simulink model "RobustFormationControl_IntegerModel_under_Dis"  (R2023a)
settings: Solver=ode3  StartTime=0.0  StopTime=30  FixedStep=0.0001  RelTol=1e-3
InitFcn:
  | % % Parameters for the fractional order NTFSMC:
  | % Sliding Surface " Sx, Sy, and Sz ":
  | %------------------------
  | % 10
  | % 10
  | cx = 2*[4 4 4];
  | cxx = 1*[0.01 0.01 0.01];
  | 
  | cx1 = cx(1);
  | cy1 = cx(2);
  | cz1 = cx(3);
  | 
  | cx2 = cxx(1);
  | cy2 = cxx(2);
  | cz2 = cxx(3);
  | 
  | alpha1 = [0.6 0.6 0.6];
  | alpha2 = [0.1 0.1 0.1];
  | 
  | gammaX = [3 3 3];
  | gx  = gammaX(1);
  | gy = gammaX(2);
  | gz = gammaX(3);
  | 
  | p = 10;
  | q = 10;
  | 
  | % Sliding Surface " S_Phi , S_Theta, and  S_Psi":
  | %------------------------
  | cP = 2*[4 4 4];
  | cPP = 1*[0.01 0.01 0.01 0.01];
  | 
  | cPhi1 = cP(1);
  | cTheta1 = cP(2);
  | cPsi1 = cP(3);
  | 
  | cPhi2 = cPP(1);
  | cTheta2 = cPP(2);
  | cPsi2 = cPP(3);
  | gammaP = [3 3 3];
  | 
  | %=========================
  | %=========================
  | SigmaX = 1*[0.01 0.01 0.01];
  | SigmaXX =1*[1 1 1];
  | 
  | Sigma1X = SigmaX(1);
  | Sigma1Y = SigmaX(2);
  | Sigma1Z = SigmaX(3);
  | %-----
  | Sigma2X = SigmaXX(1);
  | Sigma2Y = SigmaXX(2);
  | Sigma2Z = SigmaXX(3);
  | 
  | 
  | SigmaP = 1*[0.01 0.01 0.01];
  | SigmaPP =1*[1 1 1];
  | 
  | Sigma1Phi   = SigmaP(1);
  | Sigma1Theta = SigmaP(2);
  | ... (+80 lines)
values from neighbouring files (symbols this model uses):
  a1 = (Iyy - Izz)/Ixx    (= -0.812397034596)    [init_quadrotor_params.m]
  a2 = (Izz - Ixx)/Iyy    (= 0.812397034596)    [init_quadrotor_params.m]
  a3 = (Ixx - Iyy)/Izz    (= 0)    [init_quadrotor_params.m]
  a4 = - Ktx/m    (= -0.00114547325103)    [init_quadrotor_params.m]
  a5 = - Kty/m    (= -0.00114547325103)    [init_quadrotor_params.m]
  a6 = - Ktz/m    (= -0.00130740740741)    [init_quadrotor_params.m]
  b = 2.980e-5    (= 2.98e-05)    [init_quadrotor_params.m]
  b1 = - Jr/Ixx    (= -0.00584534596376)    [init_quadrotor_params.m]
  b2 = Jr/Iyy    (= 0.00584534596376)    [init_quadrotor_params.m]
  b3 = - Kfz/Izz    (= -0.0721963413248)    [init_quadrotor_params.m]
  b4 = 1/m    (= 2.05761316872)    [init_quadrotor_params.m]
  b5 = 1/m    (= 2.05761316872)    [init_quadrotor_params.m]
  b6 = 1/m    (= 2.05761316872)    [init_quadrotor_params.m]
  c1 = - Kfx/Ixx    (= -0.114641680395)    [init_quadrotor_params.m]
  c2 = - Kfy/Iyy    (= -0.114641680395)    [init_quadrotor_params.m]
  c3 = 1/Izz    (= 113.62345188)    [init_quadrotor_params.m]
  d = 1.12e-06    [init_quadrotor_params.m]
  d1 = L/Ixx    (= 46.334431631)    [init_quadrotor_params.m]
  d2 = L/Iyy    (= 46.334431631)    [init_quadrotor_params.m]
  g = 9.81    [init_quadrotor_params.m]
  Ixx = 4.856e-3    (= 0.004856)    [init_quadrotor_params.m]
  Iyy = 4.856e-3    (= 0.004856)    [init_quadrotor_params.m]
  Izz = 8.801e-3    (= 0.008801)    [init_quadrotor_params.m]
  Jr = 2.8385e-5    (= 2.8385e-05)    [init_quadrotor_params.m]
  Kfx = 5.567e-4    (= 0.0005567)    [init_quadrotor_params.m]
  Kfy = 5.567e-4    (= 0.0005567)    [init_quadrotor_params.m]
  Kfz = 6.354e-4    (= 0.0006354)    [init_quadrotor_params.m]
  Ktx = 5.5670e-4    (= 0.0005567)    [init_quadrotor_params.m]
  Kty = 5.5670e-4    (= 0.0005567)    [init_quadrotor_params.m]
  Ktz = 6.3540e-4    (= 0.0006354)    [init_quadrotor_params.m]
  L = 0.225    [init_quadrotor_params.m]
  m = 0.486    [init_quadrotor_params.m]
libraries: fod x120, eeStairGenerator x5
(part 5 of 9)

== system RobustFormationControl_IntegerModel_under_Dis/Integer Leader and four followers/Follower 4 System/Follower 2 Quadrotor Model/Control Module1/Subsystem5 ==
  x5 : Inport
  x2 : Inport  Port=2
  x4 : Inport  Port=3
  x6 : Inport  Port=4
  xd5 : Inport  Port=5
  xd6 : Inport  Port=6
  S6 : Inport  Port=7
  Constant : Constant
  Constant3 : Constant  Value=c3
  Derivative : Derivative
  Divide : Product  Inputs=*/
  Product2 : Product
  Subsystem : Subsystem
  Subsystem1 : Subsystem
  Subsystem2 : Subsystem
  Sum2 : Sum  Inputs=+++
  U4 : Outport  VectorParamsAs1DForOutWhenUnconnected=off
  wires:
  Constant/1 -> Divide/1
  Constant3/1 -> Divide/2
  S6/1 -> [S6]
  xd6/1 -> [xd6], Derivative/1
  Derivative/1 -> [xdDot6]
  xd5/1 -> [xd5]
  x2/1 -> [x2]
  Sum2/1 -> Product2/2
  Divide/1 -> Product2/1
  Product2/1 -> U4/1
  x4/1 -> [x4]
  x6/1 -> [x6]
  x5/1 -> [x5]
  [x5] -> Subsystem/1(x5)
  [x4] -> Subsystem1/1(x4)
  [x6] -> Subsystem1/2(x6)
  [x2] -> Subsystem1/3(x2)
  [xdDot6] -> Subsystem1/4(xd6)
  [xd5] -> Subsystem/2(xd5)
  [xd6] -> Subsystem/4(xd6)
  [x6] -> Subsystem/3(x6)
  [S6] -> Subsystem/5(S4)
  [xd5] -> Subsystem2/2(xd5)
  [S6] -> Subsystem2/5(S6)
  [x6] -> Subsystem2/3(x6)
  [x5] -> Subsystem2/1(x5)
  [xd6] -> Subsystem2/4(xd6)
  Subsystem/1(D2) -> Sum2/2
  Subsystem2/1(D3) -> Sum2/3
  Subsystem1/1(D1) -> Sum2/1

== system RobustFormationControl_IntegerModel_under_Dis/Integer Leader and four followers/Follower 4 System/Follower 2 Quadrotor Model/Control Module1/Subsystem6 ==
  U1 : Inport
  x7 : Inport  Port=2
  x8 : Inport  Port=3
  xL : Inport  Port=4
  dX : Inport  Port=5
  S8 : Inport  Port=6
  Constant1 : Constant
  Divide1 : Product  Inputs=*/
  Divide2 : Product  Inputs=**  RndMeth=Zero  SaturateOnIntegerOverflow=on
  Gain1 : Gain  Commented=on  Gain=b4
  Product2 : Product
  Subsystem3 : Subsystem
  Subsystem4 : Subsystem
  Subsystem5 : Subsystem
  Sum1 : Sum  Inputs=+++
  Ux : Outport  VectorParamsAs1DForOutWhenUnconnected=off
  wires:
  S8/1 -> [S8]
  dX/1 -> [dX]
  xL/1 -> [xL]
  Product2/1 -> Ux/1
  x7/1 -> [x7]
  x8/1 -> [x8]
  U1/1 -> [U1]
  Divide1/1 -> Product2/1
  Constant1/1 -> Divide1/1
  [b4D] -> Divide2/1
  [U1] -> Divide2/2
  Divide2/1 -> Divide1/2
  [dX] -> Subsystem4/3(dX)
  [dX] -> Subsystem3/4(dX)
  Subsystem4/1(D1) -> Sum1/1
  Subsystem5/1(D3) -> Sum1/3
  [xL] -> Subsystem5/1(xL)
  Subsystem3/1(D2) -> Sum1/2
  [dX] -> Subsystem5/4(dX)
  [x7] -> Subsystem3/2(x7)
  [xL] -> Subsystem3/1(xL)
  [xL] -> Subsystem4/2(xL)
  [S8] -> Subsystem3/5(S8)
  [x7] -> Subsystem5/2(x7)
  [x8] -> Subsystem5/3(x8)
  [x8] -> Subsystem4/1(x8)
  [x8] -> Subsystem3/3(x8)
  [S8] -> Subsystem5/5(S8)
  Sum1/1 -> Product2/2

== system RobustFormationControl_IntegerModel_under_Dis/Integer Leader and four followers/Follower 4 System/Follower 2 Quadrotor Model/Control Module1/Subsystem8 ==
  x3 : Inport
  x2 : Inport  Port=2
  x4 : Inport  Port=3
  x6 : Inport  Port=4
  xd3 : Inport  Port=5
  xd4 : Inport  Port=6
  S4 : Inport  Port=7
  Omega : Inport  Port=8
  Constant : Constant
  Constant3 : Constant  Value=d2
  Derivative : Derivative
  Divide : Product  Inputs=*/
  Product2 : Product
  Subsystem : Subsystem
  Subsystem1 : Subsystem
  Subsystem2 : Subsystem
  Sum2 : Sum  Inputs=+++
  U3 : Outport  VectorParamsAs1DForOutWhenUnconnected=off
  wires:
  Constant/1 -> Divide/1
  Constant3/1 -> Divide/2
  S4/1 -> [S4]
  xd4/1 -> [xd4], Derivative/1
  Derivative/1 -> [xdDot4]
  xd3/1 -> [xd3]
  x2/1 -> [x2]
  Sum2/1 -> Product2/2
  Divide/1 -> Product2/1
  Product2/1 -> U3/1
  x4/1 -> [x4]
  x6/1 -> [x6]
  x3/1 -> [x3]
  [x3] -> Subsystem/1(x3)
  [x4] -> Subsystem1/1(x4)
  [x6] -> Subsystem1/2(x6)
  [x2] -> Subsystem1/3(x2)
  Omega/1 -> Subsystem1/4(Omega)
  [xdDot4] -> Subsystem1/5(xd4)
  [xd3] -> Subsystem/2(xd3)
  [xd4] -> Subsystem/4(xd4)
  [x4] -> Subsystem/3(x4)
  [S4] -> Subsystem/5(S4)
  [xd3] -> Subsystem2/2(xd3)
  [S4] -> Subsystem2/5(S4)
  [x4] -> Subsystem2/3(x4)
  [x3] -> Subsystem2/1(x3)
  [xd4] -> Subsystem2/4(xd4)
  Subsystem/1(D2) -> Sum2/2
  Subsystem2/1(D3) -> Sum2/3
  Subsystem1/1(D1) -> Sum2/1

== system RobustFormationControl_IntegerModel_under_Dis/Integer Leader and four followers/Follower 4 System/Follower 2 Quadrotor Model/Quadrotor Dynamic System/Rotational System ==
  U2 : Inport
  U3 : Inport  Port=2
  U4 : Inport  Port=3
  Omega : Inport  Port=4
  Equation1 : Subsystem
  Equation2 : Subsystem
  Equation3 : Subsystem
  Phi or x1 : Outport  VectorParamsAs1DForOutWhenUnconnected=off
  Theta or x3 : Outport  Port=2  VectorParamsAs1DForOutWhenUnconnected=off
  Psi or x5 : Outport  Port=3  VectorParamsAs1DForOutWhenUnconnected=off
  x2 : Outport  Port=4  VectorParamsAs1DForOutWhenUnconnected=off
  x4 : Outport  Port=5  VectorParamsAs1DForOutWhenUnconnected=off
  x6 : Outport  Port=6  VectorParamsAs1DForOutWhenUnconnected=off
  wires:
  Equation1/1(x1 = Phi) -> Phi or x1/1
  Equation3/1(x5 =Psi) -> Psi or x5/1
  U2/1 -> Equation1/3(U2)
  U3/1 -> Equation2/3(U3)
  Equation3/2(x6) -> Equation2/2(x6), x6/1, Equation1/2(x6)
  Equation2/1(x3 =Theta) -> Theta or x3/1
  U4/1 -> Equation3/3(U4)
  Omega/1 -> Equation2/4(Omega), Equation1/4(Omega)
  Equation1/2(x2) -> x2/1, Equation2/1(x2), Equation3/1(x2)
  Equation2/2(x4) -> x4/1, Equation3/2(x4), Equation1/1(x4)

== system RobustFormationControl_IntegerModel_under_Dis/Integer Leader and four followers/Follower 4 System/Follower 2 Quadrotor Model/Quadrotor Dynamic System/Translational System ==
  U1 : Inport
  Ux : Inport  Port=2
  Uy : Inport  Port=3
  x1 : Inport  Port=4
  x3 : Inport  Port=5
  Equation4 : Subsystem
  Equation5 : Subsystem
  Equation6 : Subsystem
  x or x7 : Outport  VectorParamsAs1DForOutWhenUnconnected=off
  y or x9 : Outport  Port=2  VectorParamsAs1DForOutWhenUnconnected=off
  z or x11 : Outport  Port=3  VectorParamsAs1DForOutWhenUnconnected=off
  xdot or x8 : Outport  Port=4  VectorParamsAs1DForOutWhenUnconnected=off
  ydot or x10 : Outport  Port=5  VectorParamsAs1DForOutWhenUnconnected=off
  zdot or x12 : Outport  Port=6  VectorParamsAs1DForOutWhenUnconnected=off
  wires:
  Ux/1 -> Equation4/2(Ux)
  Uy/1 -> Equation5/2(Uy)
  x1/1 -> Equation6/2(x1)
  x3/1 -> Equation6/3(x3)
  Equation5/1(x9 = y) -> y or x9/1
  Equation6/1(x11 = z) -> z or x11/1
  Equation4/1(x7 = x) -> x or x7/1
  U1/1 -> Equation6/1(U1), Equation5/1(U1), Equation4/1(U1)
  Equation4/2(x8 = xdot) -> xdot or x8/1
  Equation5/2(x10 = ydot) -> ydot or x10/1
  Equation6/2(x12 = zdot) -> zdot or x12/1

== system RobustFormationControl_IntegerModel_under_Dis/Integer Leader and four followers/Leader System/Integer Model/Control Module1/Desired System ==
  Phi_d : Inport
  Theta_d : Inport  Port=2
  Psi_d : Inport  Port=3
  xd : Inport  Port=4
  yd : Inport  Port=5
  zd : Inport  Port=6
  Derivative{,1..5} (6 alike) : Derivative
  xd1 : Outport  VectorParamsAs1DForOutWhenUnconnected=off
  xd2 : Outport  Port=2  VectorParamsAs1DForOutWhenUnconnected=off
  xd3 : Outport  Port=3  VectorParamsAs1DForOutWhenUnconnected=off
  xd4 : Outport  Port=4  VectorParamsAs1DForOutWhenUnconnected=off
  xd5 : Outport  Port=5  VectorParamsAs1DForOutWhenUnconnected=off
  xd6 : Outport  Port=6  VectorParamsAs1DForOutWhenUnconnected=off
  xd7 : Outport  Port=7  VectorParamsAs1DForOutWhenUnconnected=off
  xd8 : Outport  Port=8  VectorParamsAs1DForOutWhenUnconnected=off
  xd9 : Outport  Port=9  VectorParamsAs1DForOutWhenUnconnected=off
  xd10 : Outport  Port=10  VectorParamsAs1DForOutWhenUnconnected=off
  xd11 : Outport  Port=11  VectorParamsAs1DForOutWhenUnconnected=off
  xd12 : Outport  Port=12  VectorParamsAs1DForOutWhenUnconnected=off
  wires:
  Phi_d/1 -> Derivative/1, xd1/1
  Derivative/1 -> xd2/1
  Derivative1/1 -> xd4/1
  Theta_d/1 -> Derivative1/1, xd3/1
  Psi_d/1 -> Derivative2/1, xd5/1
  Derivative2/1 -> xd6/1
  Derivative3/1 -> xd8/1
  Derivative4/1 -> xd10/1
  Derivative5/1 -> xd12/1
  xd/1 -> Derivative3/1, xd7/1
  yd/1 -> Derivative4/1, xd9/1
  zd/1 -> Derivative5/1, xd11/1

== system RobustFormationControl_IntegerModel_under_Dis/Integer Leader and four followers/Leader System/Integer Model/Control Module1/Omega Equations ==
  U1 : Inport
  U2 : Inport  Port=2
  U3 : Inport  Port=3
  U4 : Inport  Port=4
  Add1 : Sum  Inputs=+--
  Add2 : Sum  Inputs=+++
  Add3 : Sum  Inputs=++-
  Add5 : Sum  Inputs=+-+
  Control Inputs : Subsystem
  Gain11 : Gain  Gain=1/(4*b)
  Gain12 : Gain  Gain=1/(4*d)
  Gain7 : Gain  Gain=1/(2*b)
  Gain8 : Gain  Gain=1/(2*b)
  Omega : Outport  VectorParamsAs1DForOutWhenUnconnected=off
  wires:
  Add5/1 -> Control Inputs/1(w1_sqt)
  Add1/1 -> Control Inputs/2(w2_sqt)
  Add2/1 -> Control Inputs/3(w3_sqt)
  Gain11/1 -> Add5/1, Add3/1, Add2/1, Add1/1
  Gain12/1 -> Add5/3, Add2/3, Add3/3, Add1/3
  Gain7/1 -> Add5/2, Add2/2
  Gain8/1 -> Add3/2, Add1/2
  U4/1 -> Gain12/1
  U1/1 -> Gain11/1
  U3/1 -> Gain7/1
  U2/1 -> Gain8/1
  Add3/1 -> Control Inputs/4(w4_sqt)
  Control Inputs/1(Omega) -> Omega/1

== system RobustFormationControl_IntegerModel_under_Dis/Integer Leader and four followers/Leader System/Integer Model/Control Module1/Subsystem ==
  Ux : Inport
  Uy : Inport  Port=2
  Psi_d : Inport  Port=3
  Subsystem : Subsystem
  Subsystem1 : Subsystem
  Phi_d : Outport  VectorParamsAs1DForOutWhenUnconnected=off
  Theta_d : Outport  Port=2  VectorParamsAs1DForOutWhenUnconnected=off
  wires:
  Ux/1 -> Subsystem1/1(Ux), Subsystem/1(Ux)
  Uy/1 -> Subsystem1/2(Uy), Subsystem/2(Uy)
  Psi_d/1 -> Subsystem1/3(Psi_d), Subsystem/3(Psi_d)
  Subsystem/1(Phi_d) -> Subsystem1/4(Phi_d), Phi_d/1
  Subsystem1/1(Theta_d) -> Theta_d/1

== system RobustFormationControl_IntegerModel_under_Dis/Integer Leader and four followers/Leader System/Integer Model/Control Module1/Subsystem1 ==
  x1 : Inport
  x2 : Inport  Port=2
  x3 : Inport  Port=3
  x4 : Inport  Port=4
  x5 : Inport  Port=5
  x6 : Inport  Port=6
  x7 : Inport  Port=7
  x8 : Inport  Port=8
  x9 : Inport  Port=9
  x10 : Inport  Port=10
  x11 : Inport  Port=11
  x12 : Inport  Port=12
  xd1 : Inport  Port=13
  xd2 : Inport  Port=14
  xd3 : Inport  Port=15
  xd4 : Inport  Port=16
  xd5 : Inport  Port=17
  xd6 : Inport  Port=18
  xd7 : Inport  Port=19
  xd8 : Inport  Port=20
  xd9 : Inport  Port=21
  xd10 : Inport  Port=22
  xd11 : Inport  Port=23
  xd12 : Inport  Port=24
  Subsystem : Subsystem
  Subsystem1 : Subsystem
  Subsystem2 : Subsystem
  Subsystem3 : Subsystem
  Subsystem4 : Subsystem
  Subsystem6 : Subsystem
  S2 : Outport  VectorParamsAs1DForOutWhenUnconnected=off
  S4 : Outport  Port=2  VectorParamsAs1DForOutWhenUnconnected=off
  S6 : Outport  Port=3  VectorParamsAs1DForOutWhenUnconnected=off
  S8 : Outport  Port=4  VectorParamsAs1DForOutWhenUnconnected=off
  S10 : Outport  Port=5  VectorParamsAs1DForOutWhenUnconnected=off
  S12 : Outport  Port=6  VectorParamsAs1DForOutWhenUnconnected=off
  wires:
  x1/1 -> [x1]
  x2/1 -> [x2]
  x3/1 -> [x3]
  x4/1 -> [x4]
  x5/1 -> [x5]
  x6/1 -> [x6]
  x7/1 -> [x7]
  x8/1 -> [x8]
  x9/1 -> [x9]
  x10/1 -> [x10]
  x11/1 -> [x11]
  x12/1 -> [x12]
  xd1/1 -> [xd1]
  xd10/1 -> [xd10]
  xd2/1 -> [xd2]
  xd3/1 -> [xd3]
  xd4/1 -> [xd4]
  xd5/1 -> [xd5]
  xd6/1 -> [xd6]
  xd7/1 -> [xd7]
  xd8/1 -> [xd8]
  xd9/1 -> [xd9]
  xd11/1 -> [xd11]
  xd12/1 -> [xd12]
  [x1] -> Subsystem/1(x1)
  [xd1] -> Subsystem/2(xd1)
  [x2] -> Subsystem/3(x2)
  [xd2] -> Subsystem/4(xd2)
  Subsystem/1(S2) -> S2/1
  [xd4] -> Subsystem6/4(xd4)
  [x3] -> Subsystem6/1(x3)
  [x4] -> Subsystem6/3(x4)
  [xd3] -> Subsystem6/2(xd3)
  [xd6] -> Subsystem1/4(xd6)
  [x5] -> Subsystem1/1(x5)
  [x6] -> Subsystem1/3(x6)
  [xd5] -> Subsystem1/2(xd5)
  Subsystem6/1(S4) -> S4/1
  Subsystem1/1(S6) -> S6/1
  [x9] -> Subsystem3/1(x9)
  [x10] -> Subsystem3/3(x10)
  [xd9] -> Subsystem3/2(xd9)
  [xd10] -> Subsystem3/4(xd10)
  [xd8] -> Subsystem2/4(xd8)
  Subsystem3/1(S10) -> S10/1
  [xd11] -> Subsystem4/2(xd11)
  [x7] -> Subsystem2/1(x7)
  [x8] -> Subsystem2/3(x8)
  Subsystem4/1(S12) -> S12/1
  [xd7] -> Subsystem2/2(xd7)
  [x12] -> Subsystem4/3(x12)
  Subsystem2/1(S8) -> S8/1
  [xd12] -> Subsystem4/4(xd12)
  [x11] -> Subsystem4/1(x11)

== system RobustFormationControl_IntegerModel_under_Dis/Integer Leader and four followers/Leader System/Integer Model/Control Module1/Subsystem2 ==
  U1 : Inport
  x7 : Inport  Port=2
  x8 : Inport  Port=3
  xd7 : Inport  Port=4
  xd8 : Inport  Port=5
  S8 : Inport  Port=6
  Constant1 : Constant
  Derivative : Derivative
  Divide1 : Product  Inputs=*/
  Divide2 : Product  Inputs=**  RndMeth=Zero  SaturateOnIntegerOverflow=on
  Gain1 : Gain  Commented=on  Gain=b4
  Product2 : Product
  Subsystem : Subsystem
  Subsystem1 : Subsystem
  Subsystem2 : Subsystem
  Sum2 : Sum  Inputs=+++
  Ux : Outport  VectorParamsAs1DForOutWhenUnconnected=off
  wires:
  S8/1 -> [S8]
  xd8/1 -> [xd8], Derivative/1
  Derivative/1 -> [xdDot8]
  xd7/1 -> [xd7]
  Sum2/1 -> Product2/2
  Product2/1 -> Ux/1
  x7/1 -> [x7]
  x8/1 -> [x8]
  U1/1 -> [U1]
  [x7] -> Subsystem/1(x7)
  [x8] -> Subsystem1/1(x8)
  [xdDot8] -> Subsystem1/2(x8d)
  [xd7] -> Subsystem/2(xd7)
  [xd8] -> Subsystem/4(xd8)
  [x8] -> Subsystem/3(x8)
  [S8] -> Subsystem/5(S8)
  [xd7] -> Subsystem2/2(xd7)
  [S8] -> Subsystem2/5(S8)
  [x8] -> Subsystem2/3(x8)
  [x7] -> Subsystem2/1(x7)
  [xd8] -> Subsystem2/4(xd8)
  Subsystem/1(D2) -> Sum2/2
  Subsystem2/1(D3) -> Sum2/3
  Subsystem1/1(D1) -> Sum2/1
  Divide1/1 -> Product2/1
  Constant1/1 -> Divide1/1
  [b4D] -> Divide2/1
  [U1] -> Divide2/2
  Divide2/1 -> Divide1/2

== system RobustFormationControl_IntegerModel_under_Dis/Integer Leader and four followers/Leader System/Integer Model/Control Module1/Subsystem3 ==
  U1 : Inport
  x9 : Inport  Port=2
  x10 : Inport  Port=3
  xd9 : Inport  Port=4
  xd10 : Inport  Port=5
  S10 : Inport  Port=6
  Constant1 : Constant
  Derivative : Derivative
  Divide1 : Product  Inputs=*/
  Divide2 : Product  Inputs=**  RndMeth=Zero  SaturateOnIntegerOverflow=on
  Gain1 : Gain  Commented=on  Gain=b5
  Product2 : Product
  Subsystem : Subsystem
  Subsystem1 : Subsystem
  Subsystem2 : Subsystem
  Sum2 : Sum  Inputs=+++
  Uy : Outport  VectorParamsAs1DForOutWhenUnconnected=off
  wires:
  S10/1 -> [S10]
  xd10/1 -> [xd10], Derivative/1
  Derivative/1 -> [xdDot10]
  xd9/1 -> [xd9]
  Sum2/1 -> Product2/2
  Product2/1 -> Uy/1
  x9/1 -> [x9]
  x10/1 -> [x10]
  U1/1 -> [U1]
  [x9] -> Subsystem/1(x9)
  [x10] -> Subsystem1/1(x10)
  [xdDot10] -> Subsystem1/2(x10d)
  [xd9] -> Subsystem/2(xd9)
  [xd10] -> Subsystem/4(xd10)
  [x10] -> Subsystem/3(x10)
  [S10] -> Subsystem/5(S10)
  [xd9] -> Subsystem2/2(xd9)
  [S10] -> Subsystem2/5(S10)
  [x10] -> Subsystem2/3(x10)
  [x9] -> Subsystem2/1(x9)
  [xd10] -> Subsystem2/4(xd10)
  Subsystem/1(D2) -> Sum2/2
  Subsystem2/1(D3) -> Sum2/3
  Subsystem1/1(D1) -> Sum2/1
  Divide1/1 -> Product2/1
  [U1] -> Divide2/2
  Constant1/1 -> Divide1/1
  Divide2/1 -> Divide1/2
  [b5D] -> Divide2/1

== system RobustFormationControl_IntegerModel_under_Dis/Integer Leader and four followers/Leader System/Integer Model/Control Module1/Subsystem4 ==
  x1 : Inport
  x2 : Inport  Port=2
  x4 : Inport  Port=3
  x6 : Inport  Port=4
  xd1 : Inport  Port=5
  xd2 : Inport  Port=6
  S2 : Inport  Port=7
  Omega : Inport  Port=8
  Constant : Constant
  Constant3 : Constant  Commented=on  Value=d1
  Derivative : Derivative
  Divide : Product  Inputs=*/
  Product2 : Product
  Subsystem : Subsystem
  Subsystem1 : Subsystem
  Subsystem2 : Subsystem
  Sum2 : Sum  Inputs=+++
  U2 : Outport  VectorParamsAs1DForOutWhenUnconnected=off
  wires:
  Constant/1 -> Divide/1
  [d1D] -> Divide/2
  S2/1 -> [S2]
  xd2/1 -> [xd2], Derivative/1
  Derivative/1 -> [xdDot2]
  xd1/1 -> [xd1]
  x2/1 -> [x2]
  Sum2/1 -> Product2/2
  Divide/1 -> Product2/1
  Product2/1 -> U2/1
  x4/1 -> [x4]
  x6/1 -> [x6]
  x1/1 -> [x1]
  [x1] -> Subsystem/1(x1)
  [x4] -> Subsystem1/1(x4)
  [x6] -> Subsystem1/2(x6)
  [x2] -> Subsystem1/3(x2)
  Omega/1 -> Subsystem1/4(Omega)
  [xdDot2] -> Subsystem1/5(xd2)
  [xd1] -> Subsystem/2(xd1)
  [xd2] -> Subsystem/4(xd2)
  [x2] -> Subsystem/3(x2)
  [S2] -> Subsystem/5(S2)
  [xd1] -> Subsystem2/2(xd1)
  [S2] -> Subsystem2/5(S2)
  [x2] -> Subsystem2/3(x2)
  [x1] -> Subsystem2/1(x1)
  [xd2] -> Subsystem2/4(xd2)
  Subsystem1/1(D1) -> Sum2/1
  Subsystem/1(D2) -> Sum2/2
  Subsystem2/1(D3) -> Sum2/3

== system RobustFormationControl_IntegerModel_under_Dis/Integer Leader and four followers/Leader System/Integer Model/Control Module1/Subsystem5 ==
  x5 : Inport
  x2 : Inport  Port=2
  x4 : Inport  Port=3
  x6 : Inport  Port=4
  xd5 : Inport  Port=5
  xd6 : Inport  Port=6
  S6 : Inport  Port=7
  Constant : Constant
  Constant3 : Constant  Commented=on  Value=c3
  Derivative : Derivative
  Divide : Product  Inputs=*/
  Product2 : Product
  Subsystem : Subsystem
  Subsystem1 : Subsystem
  Subsystem2 : Subsystem
  Sum2 : Sum  Inputs=+++
  U4 : Outport  VectorParamsAs1DForOutWhenUnconnected=off
  wires:
  Constant/1 -> Divide/1
  [c3D] -> Divide/2
  S6/1 -> [S6]
  xd6/1 -> [xd6], Derivative/1
  Derivative/1 -> [xdDot6]
  xd5/1 -> [xd5]
  x2/1 -> [x2]
  Sum2/1 -> Product2/2
  Divide/1 -> Product2/1
  Product2/1 -> U4/1
  x4/1 -> [x4]
  x6/1 -> [x6]
  x5/1 -> [x5]
  [x5] -> Subsystem/1(x5)
  [x4] -> Subsystem1/1(x4)
  [x6] -> Subsystem1/2(x6)
  [x2] -> Subsystem1/3(x2)
  [xdDot6] -> Subsystem1/4(xd6)
  [xd5] -> Subsystem/2(xd5)
  [xd6] -> Subsystem/4(xd6)
  [x6] -> Subsystem/3(x6)
  [S6] -> Subsystem/5(S4)
  [xd5] -> Subsystem2/2(xd5)
  [S6] -> Subsystem2/5(S6)
  [x6] -> Subsystem2/3(x6)
  [x5] -> Subsystem2/1(x5)
  [xd6] -> Subsystem2/4(xd6)
  Subsystem/1(D2) -> Sum2/2
  Subsystem2/1(D3) -> Sum2/3
  Subsystem1/1(D1) -> Sum2/1

== system RobustFormationControl_IntegerModel_under_Dis/Integer Leader and four followers/Leader System/Integer Model/Control Module1/Subsystem6 ==
  x1 : Inport
  x3 : Inport  Port=2
  x11 : Inport  Port=3
  x12 : Inport  Port=4
  xd11 : Inport  Port=5
  xd12 : Inport  Port=6
  S12 : Inport  Port=7
  Constant1 : Constant
  Derivative : Derivative
  Divide1 : Product  Inputs=*/
  Divide2 : Product  Inputs=**  RndMeth=Zero  SaturateOnIntegerOverflow=on
  Gain : Gain  Commented=on  Gain=b6
  Product1 : Product
  Product2 : Product
  Subsystem : Subsystem
  Subsystem1 : Subsystem
  Subsystem2 : Subsystem
  Sum2 : Sum  Inputs=+++
  Trigonometric Function1 : Trigonometry  Operator=cos
  Trigonometric Function2 : Trigonometry  Operator=cos
  U1 : Outport  VectorParamsAs1DForOutWhenUnconnected=off
  wires:
  S12/1 -> [S12]
  xd12/1 -> [xd12], Derivative/1
  Derivative/1 -> [xdDot12]
  xd11/1 -> [xd11]
  x3/1 -> [x3]
  Sum2/1 -> Product2/2
  Product2/1 -> U1/1
  x11/1 -> [x11]
  x12/1 -> [x12]
  x1/1 -> [x1]
  [x11] -> Subsystem/1(x11)
  [x12] -> Subsystem1/1(x12)
  [xdDot12] -> Subsystem1/2(x12d)
  [xd11] -> Subsystem/2(xd11)
  [xd12] -> Subsystem/4(xd12)
  [x12] -> Subsystem/3(x12)
  [S12] -> Subsystem/5(S12)
  [xd11] -> Subsystem2/2(xd11)
  [S12] -> Subsystem2/5(S12)
  [x12] -> Subsystem2/3(x12)
  [x11] -> Subsystem2/1(x11)
  [xd12] -> Subsystem2/4(xd12)
  Subsystem/1(D2) -> Sum2/2
  Subsystem2/1(D3) -> Sum2/3
  Subsystem1/1(D1) -> Sum2/1
  Divide1/1 -> Product2/1
  Constant1/1 -> Divide1/1
  Trigonometric Function2/1 -> Product1/2
  Trigonometric Function1/1 -> Product1/1
  Divide2/1 -> Divide1/2
  Product1/1 -> Divide2/2
  [x1] -> Trigonometric Function1/1
  [x3] -> Trigonometric Function2/1
  [b6D] -> Divide2/1

== system RobustFormationControl_IntegerModel_under_Dis/Integer Leader and four followers/Leader System/Integer Model/Control Module1/Subsystem8 ==
  x3 : Inport
  x2 : Inport  Port=2
  x4 : Inport  Port=3
  x6 : Inport  Port=4
  xd3 : Inport  Port=5
  xd4 : Inport  Port=6
  S4 : Inport  Port=7
  Omega : Inport  Port=8
  Constant : Constant
  Constant3 : Constant  Commented=on  Value=d2
  Derivative : Derivative
  Divide : Product  Inputs=*/
  Product2 : Product
  Subsystem : Subsystem
  Subsystem1 : Subsystem
  Subsystem2 : Subsystem
  Sum2 : Sum  Inputs=+++
  U3 : Outport  VectorParamsAs1DForOutWhenUnconnected=off
  wires:
  Constant/1 -> Divide/1
  [d2D] -> Divide/2
  S4/1 -> [S4]
  xd4/1 -> [xd4], Derivative/1
  Derivative/1 -> [xdDot4]
  xd3/1 -> [xd3]
  x2/1 -> [x2]
  Sum2/1 -> Product2/2
  Divide/1 -> Product2/1
  Product2/1 -> U3/1
  x4/1 -> [x4]
  x6/1 -> [x6]
  x3/1 -> [x3]
  [x3] -> Subsystem/1(x3)
  [x4] -> Subsystem1/1(x4)
  [x6] -> Subsystem1/2(x6)
  [x2] -> Subsystem1/3(x2)
  Omega/1 -> Subsystem1/4(Omega)
  [xdDot4] -> Subsystem1/5(xd4)
  [xd3] -> Subsystem/2(xd3)
  [xd4] -> Subsystem/4(xd4)
  [x4] -> Subsystem/3(x4)
  [S4] -> Subsystem/5(S4)
  [xd3] -> Subsystem2/2(xd3)
  [S4] -> Subsystem2/5(S4)
  [x4] -> Subsystem2/3(x4)
  [x3] -> Subsystem2/1(x3)
  [xd4] -> Subsystem2/4(xd4)
  Subsystem/1(D2) -> Sum2/2
  Subsystem2/1(D3) -> Sum2/3
  Subsystem1/1(D1) -> Sum2/1

== system RobustFormationControl_IntegerModel_under_Dis/Integer Leader and four followers/Leader System/Integer Model/Quadrotor Dynamic System/Rotational System ==
  U2 : Inport
  U3 : Inport  Port=2
  U4 : Inport  Port=3
  Omega : Inport  Port=4
  Equation1 : Subsystem
  Equation2 : Subsystem
  Equation3 : Subsystem
  Phi or x1 : Outport  VectorParamsAs1DForOutWhenUnconnected=off
  Theta or x3 : Outport  Port=2  VectorParamsAs1DForOutWhenUnconnected=off
  Psi or x5 : Outport  Port=3  VectorParamsAs1DForOutWhenUnconnected=off
  x2 : Outport  Port=4  VectorParamsAs1DForOutWhenUnconnected=off
  x4 : Outport  Port=5  VectorParamsAs1DForOutWhenUnconnected=off
  x6 : Outport  Port=6  VectorParamsAs1DForOutWhenUnconnected=off
  wires:
  Equation1/1(x1 = Phi) -> Phi or x1/1
  Equation3/1(x5 =Psi) -> Psi or x5/1
  U2/1 -> Equation1/3(U2)
  U3/1 -> Equation2/3(U3)
  Equation3/2(x6) -> Equation2/2(x6), x6/1, Equation1/2(x6)
  Equation2/1(x3 =Theta) -> Theta or x3/1
  U4/1 -> Equation3/3(U4)
  Omega/1 -> Equation2/4(Omega), Equation1/4(Omega)
  Equation1/2(x2) -> x2/1, Equation2/1(x2), Equation3/1(x2)
  Equation2/2(x4) -> x4/1, Equation3/2(x4), Equation1/1(x4)

== system RobustFormationControl_IntegerModel_under_Dis/Integer Leader and four followers/Leader System/Integer Model/Quadrotor Dynamic System/Translational System ==
  U1 : Inport
  Ux : Inport  Port=2
  Uy : Inport  Port=3
  x1 : Inport  Port=4
  x3 : Inport  Port=5
  Equation4 : Subsystem
  Equation5 : Subsystem
  Equation6 : Subsystem
  x or x7 : Outport  VectorParamsAs1DForOutWhenUnconnected=off
  y or x9 : Outport  Port=2  VectorParamsAs1DForOutWhenUnconnected=off
  z or x11 : Outport  Port=3  VectorParamsAs1DForOutWhenUnconnected=off
  xdot or x8 : Outport  Port=4  VectorParamsAs1DForOutWhenUnconnected=off
  ydot or x10 : Outport  Port=5  VectorParamsAs1DForOutWhenUnconnected=off
  zdot or x12 : Outport  Port=6  VectorParamsAs1DForOutWhenUnconnected=off
  wires:
  Ux/1 -> Equation4/2(Ux)
  Uy/1 -> Equation5/2(Uy)
  x1/1 -> Equation6/2(x1)
  x3/1 -> Equation6/3(x3)
  Equation5/1(x9 = y) -> y or x9/1
  Equation6/1(x11 = z) -> z or x11/1
  Equation4/1(x7 = x) -> x or x7/1
  U1/1 -> Equation6/1(U1), Equation5/1(U1), Equation4/1(U1)
  Equation4/2(x8 = xdot) -> xdot or x8/1
  Equation5/2(x10 = ydot) -> ydot or x10/1
  Equation6/2(x12 = zdot) -> zdot or x12/1

== system RobustFormationControl_IntegerModel_under_Dis/Integer Leader and four followers/Follower 1 System/Follower 1 Quadrotor Model/Control Module1/Omega Equations/Control Inputs ==
  w1_sqt : Inport
  w2_sqt : Inport  Port=2
  w3_sqt : Inport  Port=3
  w4_sqt : Inport  Port=4
  Add4 : Sum  Inputs=+-+-
  Omega : Outport  VectorParamsAs1DForOutWhenUnconnected=off
  wires:
  Add4/1 -> Omega/1
  w1_sqt/1 -> Add4/1
  w2_sqt/1 -> Add4/2
  w3_sqt/1 -> Add4/3
  w4_sqt/1 -> Add4/4

== system RobustFormationControl_IntegerModel_under_Dis/Integer Leader and four followers/Follower 1 System/Follower 1 Quadrotor Model/Control Module1/Subsystem/Subsystem ==
  Ux : Inport
  Uy : Inport  Port=2
  Psi_d : Inport  Port=3
  Product : Product
  Product1 : Product
  Subtract : Sum  Inputs=+-
  Trigonometric Function : Trigonometry
  Trigonometric Function1 : Trigonometry  Operator=cos
  Trigonometric Function2 : Trigonometry  Operator=asin
  Phi_d : Outport  VectorParamsAs1DForOutWhenUnconnected=off
  wires:
  Product1/1 -> Subtract/2
  Uy/1 -> Product1/2
  Ux/1 -> Product/1
  Trigonometric Function1/1 -> Product1/1
  Psi_d/1 -> Trigonometric Function1/1, Trigonometric Function/1
  Product/1 -> Subtract/1
  Subtract/1 -> Trigonometric Function2/1
  Trigonometric Function/1 -> Product/2
  Trigonometric Function2/1 -> Phi_d/1

== system RobustFormationControl_IntegerModel_under_Dis/Integer Leader and four followers/Follower 1 System/Follower 1 Quadrotor Model/Control Module1/Subsystem/Subsystem1 ==
  Ux : Inport
  Uy : Inport  Port=2
  Psi_d : Inport  Port=3
  Phi_d : Inport  Port=4
  Constant : Constant
  Divide : Product  Inputs=*/
  Product : Product
  Product1 : Product
  Product2 : Product
  Subtract : Sum
  Trigonometric Function : Trigonometry  Operator=cos
  Trigonometric Function1 : Trigonometry
  Trigonometric Function2 : Trigonometry  Operator=asin
  Trigonometric Function3 : Trigonometry  Operator=cos
  Theta_d : Outport  VectorParamsAs1DForOutWhenUnconnected=off
  wires:
  Product1/1 -> Subtract/2
  Uy/1 -> Product1/2
  Ux/1 -> Product/1
  Trigonometric Function1/1 -> Product1/1
  Psi_d/1 -> Trigonometric Function1/1, Trigonometric Function/1
  Product/1 -> Subtract/1
  Trigonometric Function/1 -> Product/2
  Trigonometric Function2/1 -> Theta_d/1
  Constant/1 -> Divide/1
  Product2/1 -> Trigonometric Function2/1
  Subtract/1 -> Product2/1
  Divide/1 -> Product2/2
  Trigonometric Function3/1 -> Divide/2
  Phi_d/1 -> Trigonometric Function3/1

== system RobustFormationControl_IntegerModel_under_Dis/Integer Leader and four followers/Follower 1 System/Follower 1 Quadrotor Model/Control Module1/Subsystem1/Subsystem ==
  x1 : Inport
  xd1 : Inport  Port=2
  x2 : Inport  Port=3
  xd2 : Inport  Port=4
  Constant : Constant  Value=p/q
  Constant1 : Constant  Value=gx
  Divide : Product  Inputs=**  RndMeth=Zero  SaturateOnIntegerOverflow=on
  Fractional integrator : fod/Fractional integrator  gam=alpha1(1)  ww=[0.001; 1000]  n=5  nFod=off
      settings: SourceProductName=FOMCON Toolbox
  Fractional integrator1 : fod/Fractional integrator  gam=alpha2(1)  ww=[0.001; 1000]  n=5  nFod=off
      settings: SourceProductName=FOMCON Toolbox
  Gain : Gain  Gain=cPhi1
  Gain1 : Gain  Gain=cPhi2
  Power : Math  Operator=pow
  Power1 : Math  Operator=pow
  Sign : Signum
  Sum1 : Sum  Inputs=+-
  Sum2 : Sum  Inputs=+++
  Sum3 : Sum  Inputs=+-
  S2 : Outport  VectorParamsAs1DForOutWhenUnconnected=off
  wires:
  xd2/1 -> Sum1/2
  Sum2/1 -> S2/1
  xd1/1 -> Sum3/2
  x1/1 -> Sum3/1
  x2/1 -> Sum1/1
  Sum3/1 -> Power1/1, Sign/1, Power/1
  Constant/1 -> Power/2
  Power/1 -> Gain/1
  Gain/1 -> Fractional integrator/1
  Constant1/1 -> Power1/2
  Sign/1 -> Divide/1
  Power1/1 -> Divide/2
  Divide/1 -> Gain1/1
  Gain1/1 -> Fractional integrator1/1
  Sum1/1 -> Sum2/1
  Fractional integrator/1 -> Sum2/2
  Fractional integrator1/1 -> Sum2/3

== system RobustFormationControl_IntegerModel_under_Dis/Integer Leader and four followers/Follower 1 System/Follower 1 Quadrotor Model/Control Module1/Subsystem1/Subsystem1 ==
  x5 : Inport
  xd5 : Inport  Port=2
  x6 : Inport  Port=3
  xd6 : Inport  Port=4
  Constant : Constant  Value=p/q
  Constant1 : Constant  Value=gz
  Divide : Product  Inputs=**  RndMeth=Zero  SaturateOnIntegerOverflow=on
  Fractional integrator : fod/Fractional integrator  gam=alpha1(3)  ww=[0.001; 1000]  n=5  nFod=off
      settings: SourceProductName=FOMCON Toolbox
  Fractional integrator1 : fod/Fractional integrator  gam=alpha2(3)  ww=[0.001; 1000]  n=5  nFod=off
      settings: SourceProductName=FOMCON Toolbox
  Gain : Gain  Gain=cPsi1
  Gain1 : Gain  Gain=cPsi2
  Power : Math  Operator=pow
  Power1 : Math  Operator=pow
  Sign : Signum
  Sum1 : Sum  Inputs=+-
  Sum2 : Sum  Inputs=+++
  Sum3 : Sum  Inputs=+-
  S6 : Outport  VectorParamsAs1DForOutWhenUnconnected=off
  wires:
  xd6/1 -> Sum1/2
  Sum2/1 -> S6/1
  xd5/1 -> Sum3/2
  x5/1 -> Sum3/1
  x6/1 -> Sum1/1
  Sum3/1 -> Power1/1, Sign/1, Power/1
  Constant/1 -> Power/2
  Power/1 -> Gain/1
  Gain/1 -> Fractional integrator/1
  Constant1/1 -> Power1/2
  Sign/1 -> Divide/1
  Power1/1 -> Divide/2
  Divide/1 -> Gain1/1
  Gain1/1 -> Fractional integrator1/1
  Sum1/1 -> Sum2/1
  Fractional integrator/1 -> Sum2/2
  Fractional integrator1/1 -> Sum2/3

== system RobustFormationControl_IntegerModel_under_Dis/Integer Leader and four followers/Follower 1 System/Follower 1 Quadrotor Model/Control Module1/Subsystem1/Subsystem2 ==
  yL : Inport
  x9 : Inport  Port=2
  x10 : Inport  Port=3
  dY : Inport  Port=4
  Constant : Constant  Value=p/q
  Constant1 : Constant  Value=gy
  Derivative : Derivative
  Derivative1 : Derivative
  Divide : Product  Inputs=**  RndMeth=Zero  SaturateOnIntegerOverflow=on
  Fractional integrator : fod/Fractional integrator  gam=alpha1(2)  ww=[0.001; 1000]  n=5  nFod=off
      settings: SourceProductName=FOMCON Toolbox
  Fractional integrator1 : fod/Fractional integrator  gam=alpha2(2)  ww=[0.001; 1000]  n=5  nFod=off
      settings: SourceProductName=FOMCON Toolbox
  Gain2 : Gain  Gain=cy1
  Gain3 : Gain  Gain=cy2
  Power : Math  Operator=pow
  Power1 : Math  Operator=pow
  Sign : Signum
  Sum1 : Sum  Inputs=+--
  Sum3 : Sum  Inputs=+--
  Sum5 : Sum  Inputs=+++
  S10 : Outport  VectorParamsAs1DForOutWhenUnconnected=off
  wires:
  x9/1 -> Sum3/2
  yL/1 -> Sum3/1, Derivative/1
  dY/1 -> Sum3/3, Derivative1/1
  x10/1 -> Sum1/3
  Derivative/1 -> Sum1/1
  Derivative1/1 -> Sum1/2
  Fractional integrator1/1 -> Sum5/3
  Fractional integrator/1 -> Sum5/2
  Gain3/1 -> Fractional integrator1/1
  Sum1/1 -> Sum5/1
  Sum5/1 -> S10/1
  Divide/1 -> Gain3/1
  Gain2/1 -> Fractional integrator/1
  Sign/1 -> Divide/1
  Power1/1 -> Divide/2
  Power/1 -> Gain2/1
  Constant1/1 -> Power1/2
  Sum3/1 -> Power1/1, Sign/1, Power/1
  Constant/1 -> Power/2

== system RobustFormationControl_IntegerModel_under_Dis/Integer Leader and four followers/Follower 1 System/Follower 1 Quadrotor Model/Control Module1/Subsystem1/Subsystem3 ==
  xL : Inport
  x7 : Inport  Port=2
  x8 : Inport  Port=3
  dX : Inport  Port=4
  Constant : Constant  Value=p/q
  Constant1 : Constant  Value=gx
  Derivative : Derivative
  Derivative1 : Derivative
  Divide : Product  Inputs=**  RndMeth=Zero  SaturateOnIntegerOverflow=on
  Fractional integrator : fod/Fractional integrator  gam=alpha1(1)  ww=[0.001; 1000]  n=5  nFod=off
      settings: SourceProductName=FOMCON Toolbox
  Fractional integrator1 : fod/Fractional integrator  gam=alpha2(1)  ww=[0.001; 1000]  n=5  nFod=off
      settings: SourceProductName=FOMCON Toolbox
  Gain2 : Gain  Gain=cx1
  Gain3 : Gain  Gain=cx2
  Power : Math  Operator=pow
  Power1 : Math  Operator=pow
  Sign : Signum
  Sum1 : Sum  Inputs=+--
  Sum3 : Sum  Inputs=+--
  Sum5 : Sum  Inputs=+++
  S8 : Outport  VectorParamsAs1DForOutWhenUnconnected=off
  wires:
  x7/1 -> Sum3/2
  xL/1 -> Sum3/1, Derivative/1
  dX/1 -> Sum3/3, Derivative1/1
  x8/1 -> Sum1/3
  Derivative/1 -> Sum1/1
  Derivative1/1 -> Sum1/2
  Fractional integrator1/1 -> Sum5/3
  Fractional integrator/1 -> Sum5/2
  Gain3/1 -> Fractional integrator1/1
  Sum1/1 -> Sum5/1
  Sum5/1 -> S8/1
  Divide/1 -> Gain3/1
  Gain2/1 -> Fractional integrator/1
  Sign/1 -> Divide/1
  Power1/1 -> Divide/2
  Power/1 -> Gain2/1
  Constant1/1 -> Power1/2
  Sum3/1 -> Power1/1, Sign/1, Power/1
  Constant/1 -> Power/2

== system RobustFormationControl_IntegerModel_under_Dis/Integer Leader and four followers/Follower 1 System/Follower 1 Quadrotor Model/Control Module1/Subsystem1/Subsystem4 ==
  zL : Inport
  x11 : Inport  Port=2
  x12 : Inport  Port=3
  dZ : Inport  Port=4
  Constant : Constant  Value=p/q
  Constant1 : Constant  Value=gz
  Derivative : Derivative
  Derivative1 : Derivative
  Divide : Product  Inputs=**  RndMeth=Zero  SaturateOnIntegerOverflow=on
  Fractional integrator : fod/Fractional integrator  gam=alpha1(2)  ww=[0.001; 1000]  n=5  nFod=off
      settings: SourceProductName=FOMCON Toolbox
  Fractional integrator1 : fod/Fractional integrator  gam=alpha2(2)  ww=[0.001; 1000]  n=5  nFod=off
      settings: SourceProductName=FOMCON Toolbox
  Gain2 : Gain  Gain=cz1
  Gain3 : Gain  Gain=cz2
  Power : Math  Operator=pow
  Power1 : Math  Operator=pow
  Sign : Signum
  Sum1 : Sum  Inputs=+--
  Sum3 : Sum  Inputs=+--
  Sum5 : Sum  Inputs=+++
  S12 : Outport  VectorParamsAs1DForOutWhenUnconnected=off
  wires:
  Constant/1 -> Power/2
  Sum3/1 -> Power/1, Sign/1, Power1/1
  Constant1/1 -> Power1/2
  Power/1 -> Gain2/1
  Power1/1 -> Divide/2
  Sign/1 -> Divide/1
  Gain2/1 -> Fractional integrator/1
  Divide/1 -> Gain3/1
  Sum5/1 -> S12/1
  Sum1/1 -> Sum5/1
  Gain3/1 -> Fractional integrator1/1
  Fractional integrator/1 -> Sum5/2
  Fractional integrator1/1 -> Sum5/3
  Derivative1/1 -> Sum1/2
  Derivative/1 -> Sum1/1
  x12/1 -> Sum1/3
  dZ/1 -> Derivative1/1, Sum3/3
  zL/1 -> Derivative/1, Sum3/1
  x11/1 -> Sum3/2

== system RobustFormationControl_IntegerModel_under_Dis/Integer Leader and four followers/Follower 1 System/Follower 1 Quadrotor Model/Control Module1/Subsystem1/Subsystem6 ==
  x3 : Inport
  xd3 : Inport  Port=2
  x4 : Inport  Port=3
  xd4 : Inport  Port=4
  Constant : Constant  Value=p/q
  Constant1 : Constant  Value=gy
  Divide : Product  Inputs=**  RndMeth=Zero  SaturateOnIntegerOverflow=on
  Fractional integrator : fod/Fractional integrator  gam=alpha1(2)  ww=[0.001; 1000]  n=5  nFod=off
      settings: SourceProductName=FOMCON Toolbox
  Fractional integrator1 : fod/Fractional integrator  gam=alpha2(2)  ww=[0.001; 1000]  n=5  nFod=off
      settings: SourceProductName=FOMCON Toolbox
  Gain : Gain  Gain=cTheta1
  Gain1 : Gain  Gain=cTheta2
  Power : Math  Operator=pow
  Power1 : Math  Operator=pow
  Sign : Signum
  Sum1 : Sum  Inputs=+-
  Sum2 : Sum  Inputs=+++
  Sum3 : Sum  Inputs=+-
  S4 : Outport  VectorParamsAs1DForOutWhenUnconnected=off
  wires:
  xd4/1 -> Sum1/2
  Sum2/1 -> S4/1
  xd3/1 -> Sum3/2
  x3/1 -> Sum3/1
  x4/1 -> Sum1/1
  Sum3/1 -> Power1/1, Sign/1, Power/1
  Constant/1 -> Power/2
  Power/1 -> Gain/1
  Gain/1 -> Fractional integrator/1
  Constant1/1 -> Power1/2
  Sign/1 -> Divide/1
  Power1/1 -> Divide/2
  Divide/1 -> Gain1/1
  Gain1/1 -> Fractional integrator1/1
  Sum1/1 -> Sum2/1
  Fractional integrator/1 -> Sum2/2
  Fractional integrator1/1 -> Sum2/3

== system RobustFormationControl_IntegerModel_under_Dis/Integer Leader and four followers/Follower 1 System/Follower 1 Quadrotor Model/Control Module1/Subsystem10/Subsystem ==
  zL : Inport
  x11 : Inport  Port=2
  x12 : Inport  Port=3
  dZ : Inport  Port=4
  S12 : Inport  Port=5
  Constant : Constant  Value=p/q
  Constant1 : Constant  Value=gz-1
  Derivative : Derivative
  Derivative1 : Derivative
  Divide : Product  Inputs=**  RndMeth=Zero  SaturateOnIntegerOverflow=on
  Fractional derivative : fod/Fractional derivative  gam=alpha1(3)  ww=[0.001; 1000]  n=5  nFod=off
      settings: SourceProductName=FOMCON Toolbox
  Fractional integrator1 : fod/Fractional integrator  gam=alpha2(3)  ww=[0.001; 1000]  n=5  nFod=off
      settings: SourceProductName=FOMCON Toolbox
  Gain : Gain  Gain=cz1
  Gain1 : Gain  Gain=cz2
  Gain2 : Gain  Gain=gz
  Gain3 : Gain  Gain=Sigma1Z
  Gain4 : Gain  Gain=Sigma2Z
  Power : Math  Operator=pow
  Power1 : Math  Operator=pow
  Sign : Signum
  Sum : Sum
  Sum1 : Sum  Inputs=+--
  Sum2 : Sum  Inputs=+++
  Sum3 : Sum  Inputs=+--
  D2 : Outport  VectorParamsAs1DForOutWhenUnconnected=off
  wires:
  Sum3/1 -> Power1/1, Power/1
  Constant/1 -> Power/2
  Power/1 -> Gain/1
  Gain/1 -> Fractional derivative/1
  Constant1/1 -> Power1/2
  Power1/1 -> Divide/2
  Divide/1 -> Gain1/1
  Gain1/1 -> Gain2/1
  Sum1/1 -> Divide/1
  Gain2/1 -> Fractional integrator1/1
  S12/1 -> Gain4/1, Sign/1
  Sign/1 -> Gain3/1
  Gain3/1 -> Sum/1
  Gain4/1 -> Sum/2
  Sum/1 -> Sum2/3
  Fractional derivative/1 -> Sum2/1
  Fractional integrator1/1 -> Sum2/2
  Sum2/1 -> D2/1
  zL/1 -> Sum3/1, Derivative/1
  Derivative/1 -> Sum1/1
  x12/1 -> Sum1/2
  dZ/1 -> Sum3/3, Derivative1/1
  Derivative1/1 -> Sum1/3
  x11/1 -> Sum3/2

== system RobustFormationControl_IntegerModel_under_Dis/Integer Leader and four followers/Follower 1 System/Follower 1 Quadrotor Model/Control Module1/Subsystem10/Subsystem1 ==
  x12 : Inport
  zL : Inport  Port=2
  dZ : Inport  Port=3
  Constant2 : Constant  Value=g
  Derivative{,1..3} (4 alike) : Derivative
  Divide2 : Product  Inputs=**  RndMeth=Zero  SaturateOnIntegerOverflow=on
  Gain1 : Gain  Commented=on  Gain=a6
  Sum : Sum  Inputs=-++-
  D1 : Outport
  wires:
  Sum/1 -> D1/1
  x12/1 -> Divide2/2
  Divide2/1 -> Sum/1
  Constant2/1 -> Sum/2
  [a6D] -> Divide2/1
  Derivative/1 -> Derivative1/1
  Derivative1/1 -> Sum/3
  zL/1 -> Derivative/1
  Derivative3/1 -> Sum/4
  Derivative2/1 -> Derivative3/1
  dZ/1 -> Derivative2/1

== system RobustFormationControl_IntegerModel_under_Dis/Integer Leader and four followers/Follower 1 System/Follower 1 Quadrotor Model/Control Module1/Subsystem10/Subsystem2 ==
  zL : Inport
  x11 : Inport  Port=2
  x12 : Inport  Port=3
  dZ : Inport  Port=4
  S12 : Inport  Port=5
  Abs : Abs  SaturateOnIntegerOverflow=off
  Derivative : Derivative
  Derivative1 : Derivative
  Divide{,1..4} (5 alike) : Product  Inputs=**  RndMeth=Zero  SaturateOnIntegerOverflow=on
  Gain : Gain  Gain=q0
  Gain1 : Gain  Gain=q1
  Gain2 : Gain  Gain=q2
  Integrator : Integrator
  Integrator1 : Integrator
  Integrator2 : Integrator
  Mux : Mux  Inputs=3
  Sign : Signum
  Sum2 : Sum  Inputs=++++
  Sum4 : Sum  Inputs=+--
  Sum5 : Sum  Inputs=+--
  To Workspace : ToWorkspace  VariableName=BzF1  SampleTime=-1
  w : Constant  Value=w
  D3 : Outport  VectorParamsAs1DForOutWhenUnconnected=off
  wires:
  S12/1 -> [S12], Abs/1
  Gain/1 -> Integrator/1
  [e1] -> Divide/2
  Gain1/1 -> Integrator1/1
  Divide/1 -> Gain1/1
  Divide1/1 -> Gain2/1
  Gain2/1 -> Integrator2/1
  [e2] -> Divide1/2
  Abs/1 -> Divide1/1, Divide/1, Gain/1
  Integrator1/1 -> Divide3/2  "B1"
  w/1 -> Sum2/4
  Sign/1 -> Divide2/2
  [S12] -> Sign/1
  Divide2/1 -> D3/1
  [e1] -> Divide3/1
  [e2] -> Divide4/1
  Integrator2/1 -> Divide4/2  "B2"
  Sum2/1 -> Divide2/1
  Derivative1/1 -> Sum4/3
  Derivative/1 -> Sum4/1
  Sum4/1 -> [e2]
  Sum5/1 -> [e1]
  zL/1 -> Sum5/1, Derivative/1
  x12/1 -> Sum4/2
  dZ/1 -> Sum5/3, Derivative1/1
  x11/1 -> Sum5/2
  Divide3/1 -> Mux/2, Sum2/2
  Divide4/1 -> Mux/3, Sum2/3
  Mux/1 -> To Workspace/1
  Integrator/1 -> Mux/1, Sum2/1  "B0"

== system RobustFormationControl_IntegerModel_under_Dis/Integer Leader and four followers/Follower 1 System/Follower 1 Quadrotor Model/Control Module1/Subsystem2/Subsystem3 ==
  yL : Inport
  x9 : Inport  Port=2
  x10 : Inport  Port=3
  dY : Inport  Port=4
  S10 : Inport  Port=5
  Constant : Constant  Value=p/q
  Constant1 : Constant  Value=gy-1
  Derivative : Derivative
  Derivative1 : Derivative
  Divide : Product  Inputs=**  RndMeth=Zero  SaturateOnIntegerOverflow=on
  Fractional derivative : fod/Fractional derivative  gam=alpha1(2)  ww=[0.001; 1000]  n=5  nFod=off
      settings: SourceProductName=FOMCON Toolbox
  Fractional integrator1 : fod/Fractional integrator  gam=alpha2(2)  ww=[0.001; 1000]  n=5  nFod=off
      settings: SourceProductName=FOMCON Toolbox
  Gain : Gain  Gain=cy1
  Gain1 : Gain  Gain=cy2
  Gain2 : Gain  Gain=gy
  Gain3 : Gain  Gain=Sigma1Y
  Gain4 : Gain  Gain=Sigma2Y
  Power : Math  Operator=pow
  Power1 : Math  Operator=pow
  Sign : Signum
  Sum : Sum
  Sum1 : Sum  Inputs=+--
  Sum2 : Sum  Inputs=+++
  Sum3 : Sum  Inputs=+--
  D2 : Outport  VectorParamsAs1DForOutWhenUnconnected=off
  wires:
  Sum3/1 -> Power1/1, Power/1
  Constant/1 -> Power/2
  Power/1 -> Gain/1
  Gain/1 -> Fractional derivative/1
  Constant1/1 -> Power1/2
  Power1/1 -> Divide/2
  Divide/1 -> Gain1/1
  Gain1/1 -> Gain2/1
  Sum1/1 -> Divide/1
  Gain2/1 -> Fractional integrator1/1
  S10/1 -> Gain4/1, Sign/1
  Sign/1 -> Gain3/1
  Gain3/1 -> Sum/1
  Gain4/1 -> Sum/2
  Sum/1 -> Sum2/3
  Fractional derivative/1 -> Sum2/1
  Fractional integrator1/1 -> Sum2/2
  Sum2/1 -> D2/1
  yL/1 -> Sum3/1, Derivative/1
  Derivative/1 -> Sum1/1
  x10/1 -> Sum1/2
  dY/1 -> Sum3/3, Derivative1/1
  Derivative1/1 -> Sum1/3
  x9/1 -> Sum3/2

== system RobustFormationControl_IntegerModel_under_Dis/Integer Leader and four followers/Follower 1 System/Follower 1 Quadrotor Model/Control Module1/Subsystem2/Subsystem4 ==
  x10 : Inport
  yL : Inport  Port=2
  dY : Inport  Port=3
  Derivative{,1..3} (4 alike) : Derivative
  Divide2 : Product  Inputs=**  RndMeth=Zero  SaturateOnIntegerOverflow=on
  Gain1 : Gain  Commented=on  Gain=a5
  Sum : Sum  Inputs=-+-
  D1 : Outport
  wires:
  Sum/1 -> D1/1
  x10/1 -> Divide2/2
  Divide2/1 -> Sum/1
  [a5D] -> Divide2/1
  Derivative/1 -> Derivative1/1
  yL/1 -> Derivative/1
  Derivative3/1 -> Sum/3
  Derivative2/1 -> Derivative3/1
  dY/1 -> Derivative2/1
  Derivative1/1 -> Sum/2

== system RobustFormationControl_IntegerModel_under_Dis/Integer Leader and four followers/Follower 1 System/Follower 1 Quadrotor Model/Control Module1/Subsystem2/Subsystem5 ==
  yL : Inport
  x9 : Inport  Port=2
  x10 : Inport  Port=3
  dY : Inport  Port=4
  S10 : Inport  Port=5
  Abs : Abs  SaturateOnIntegerOverflow=off
  Derivative : Derivative
  Derivative1 : Derivative
  Divide{,1..4} (5 alike) : Product  Inputs=**  RndMeth=Zero  SaturateOnIntegerOverflow=on
  Gain : Gain  Gain=q0
  Gain1 : Gain  Gain=q1
  Gain2 : Gain  Gain=q2
  Integrator : Integrator
  Integrator1 : Integrator
  Integrator2 : Integrator
  Mux : Mux  Inputs=3
  Sign : Signum
  Sum2 : Sum  Inputs=++++
  Sum4 : Sum  Inputs=+--
  Sum5 : Sum  Inputs=+--
  To Workspace : ToWorkspace  VariableName=ByF1  SampleTime=-1
  w : Constant  Value=w
  D3 : Outport  VectorParamsAs1DForOutWhenUnconnected=off
  wires:
  S10/1 -> [S10], Abs/1
  Gain/1 -> Integrator/1
  [e1] -> Divide/2
  Gain1/1 -> Integrator1/1
  Divide/1 -> Gain1/1
  Divide1/1 -> Gain2/1
  Gain2/1 -> Integrator2/1
  [e2] -> Divide1/2
  Abs/1 -> Divide1/1, Divide/1, Gain/1
  Integrator1/1 -> Divide3/2  "B1"
  w/1 -> Sum2/4
  Sign/1 -> Divide2/2
  [S10] -> Sign/1
  Divide2/1 -> D3/1
  [e1] -> Divide3/1
  [e2] -> Divide4/1
  Integrator2/1 -> Divide4/2  "B2"
  Sum2/1 -> Divide2/1
  Derivative1/1 -> Sum4/3
  Derivative/1 -> Sum4/1
  Sum4/1 -> [e2]
  Sum5/1 -> [e1]
  yL/1 -> Sum5/1, Derivative/1
  x10/1 -> Sum4/2
  dY/1 -> Sum5/3, Derivative1/1
  x9/1 -> Sum5/2
  Integrator/1 -> Mux/1, Sum2/1  "B0"
  Divide3/1 -> Mux/2, Sum2/2
  Divide4/1 -> Mux/3, Sum2/3
  Mux/1 -> To Workspace/1

== system RobustFormationControl_IntegerModel_under_Dis/Integer Leader and four followers/Follower 1 System/Follower 1 Quadrotor Model/Control Module1/Subsystem4/Subsystem ==
  x1 : Inport
  xd1 : Inport  Port=2
  x2 : Inport  Port=3
  xd2 : Inport  Port=4
  S2 : Inport  Port=5
  Constant : Constant  Value=p/q
  Constant1 : Constant  Value=gammaP(1)-1
  Divide : Product  Inputs=**  RndMeth=Zero  SaturateOnIntegerOverflow=on
  Fractional derivative : fod/Fractional derivative  gam=alpha1(1)  ww=[0.001; 1000]  n=5  nFod=off
      settings: SourceProductName=FOMCON Toolbox
  Fractional integrator1 : fod/Fractional integrator  gam=alpha2(2)  ww=[0.001; 1000]  n=5  nFod=off
      settings: SourceProductName=FOMCON Toolbox
  Gain : Gain  Gain=cPhi1
  Gain1 : Gain  Gain=cPhi2
  Gain2 : Gain  Gain=gammaP(1)
  Gain3 : Gain  Gain=Sigma1Phi
  Gain4 : Gain  Gain=Sigma1Phi
  Power : Math  Operator=pow
  Power1 : Math  Operator=pow
  Sign : Signum
  Sum : Sum
  Sum1 : Sum  Inputs=+-
  Sum2 : Sum  Inputs=---
  Sum3 : Sum  Inputs=+-
  D2 : Outport  VectorParamsAs1DForOutWhenUnconnected=off
  wires:
  xd2/1 -> Sum1/2
  xd1/1 -> Sum3/2
  x1/1 -> Sum3/1
  x2/1 -> Sum1/1
  Sum3/1 -> Power1/1, Power/1
  Constant/1 -> Power/2
  Power/1 -> Gain/1
  Gain/1 -> Fractional derivative/1
  Constant1/1 -> Power1/2
  Power1/1 -> Divide/2
  Divide/1 -> Gain1/1
  Gain1/1 -> Gain2/1
  Sum1/1 -> Divide/1
  Gain2/1 -> Fractional integrator1/1
  S2/1 -> Gain4/1, Sign/1
  Sign/1 -> Gain3/1
  Gain3/1 -> Sum/1
  Gain4/1 -> Sum/2
  Sum/1 -> Sum2/3
  Fractional derivative/1 -> Sum2/1
  Fractional integrator1/1 -> Sum2/2
  Sum2/1 -> D2/1

== system RobustFormationControl_IntegerModel_under_Dis/Integer Leader and four followers/Follower 1 System/Follower 1 Quadrotor Model/Control Module1/Subsystem4/Subsystem1 ==
  x4 : Inport
  x6 : Inport  Port=2
  x2 : Inport  Port=3
  Omega : Inport  Port=4
  xd2 : Inport  Port=5
  Gain : Gain  Gain=a1
  Gain6 : Gain  Gain=c1
  Gain7 : Gain  Gain=b1
  Math Function : Math  Operator=square  SignedPower=on
  Product1 : Product
  Product3 : Product
  Sum3 : Sum  Inputs=---+
  D1 : Outport
  wires:
  xd2/1 -> Sum3/4
  Product1/1 -> Gain/1
  Sum3/1 -> D1/1
  Gain6/1 -> Sum3/2  "c1 x2^2"
  Gain7/1 -> Sum3/3
  Product3/1 -> Gain7/1
  Omega/1 -> Product3/2
  Math Function/1 -> Gain6/1  "x2^2"
  x4/1 -> Product3/1, Product1/1
  Gain/1 -> Sum3/1  "a1 x4 x6"
  x6/1 -> Product1/2
  x2/1 -> Math Function/1

== system RobustFormationControl_IntegerModel_under_Dis/Integer Leader and four followers/Follower 1 System/Follower 1 Quadrotor Model/Control Module1/Subsystem4/Subsystem2 ==
  x1 : Inport
  xd1 : Inport  Port=2
  x2 : Inport  Port=3
  xd2 : Inport  Port=4
  S2 : Inport  Port=5
  Abs : Abs  SaturateOnIntegerOverflow=off
  Divide{,1..4} (5 alike) : Product  Inputs=**  RndMeth=Zero  SaturateOnIntegerOverflow=on
  Gain : Gain  Gain=q0
  Gain1 : Gain  Gain=q1
  Gain2 : Gain  Gain=q2
  Integrator : Integrator
  Integrator1 : Integrator
  Integrator2 : Integrator
  Sign : Signum
  Sum1 : Sum  Inputs=+-
  Sum2 : Sum  Inputs=----
  Sum3 : Sum  Inputs=+-
  w : Constant  Value=w
  D3 : Outport  VectorParamsAs1DForOutWhenUnconnected=off
  wires:
  xd2/1 -> Sum1/2
  xd1/1 -> Sum3/2
  x1/1 -> Sum3/1
  x2/1 -> Sum1/1
  S2/1 -> [S2], Abs/1
  Sum1/1 -> [e2]
  Sum3/1 -> [e1]
  Gain/1 -> Integrator/1
  Integrator/1 -> Sum2/1  "B0"
  [e1] -> Divide/2
  Gain1/1 -> Integrator1/1
  Divide/1 -> Gain1/1
  Divide1/1 -> Gain2/1
  Gain2/1 -> Integrator2/1
  [e2] -> Divide1/2
  Abs/1 -> Divide1/1, Divide/1, Gain/1
  Integrator1/1 -> Divide3/2  "B1"
  w/1 -> Sum2/4
  Sign/1 -> Divide2/2
  [S2] -> Sign/1
  Divide2/1 -> D3/1
  [e1] -> Divide3/1
  [e2] -> Divide4/1
  Integrator2/1 -> Divide4/2  "B2"
  Divide3/1 -> Sum2/2
  Divide4/1 -> Sum2/3
  Sum2/1 -> Divide2/1
